simulink model "MissileMathSim"  (R2025a)
settings: Solver=ode4  StartTime=0.0  StopTime=inf  FixedStep=0.01  RelTol=1e-3
values from neighbouring files (symbols this model uses):
  phi00 = [0 0.5 1 1.5 2 2.5 3 3.5 4 4.5 5 5.5 ... (552 elements, 276x2)]    [pre-design_data.mat]
libraries: slpidlib x2, ASEToolBox x1, simulink x1
settings Model: Creator=admin  LastModifiedBy=zqhkd
settings DataIOCC: SaveFinalState=on  SaveOutput=off  InspectSignalLogs=on  SaveTime=off
settings OptimizationCC: DefaultParameterBehavior=Inlined  EnhancedBackFolding=on  PassReuseOutputArgsAs=Individual arguments  ZeroExternalMemoryAtStartup=off  ZeroInternalMemoryAtStartup=off  OptimizeBlockOrder=speed  DifferentSizesBufferReuse=on  OptimizationCustomize=off  EfficientTunableParamExpr=on
settings DebuggingCC: ParameterTunabilityLossMsg=error
settings HardwareCC: ProdBitPerLong=64.0  ProdHWDeviceType=Intel->x86-64 (Linux 64)
settings SFSimCC: MATLABDynamicMemAlloc=off
settings RTWCC: SystemTargetFile=ert.tlc  TemplateMakefile=ert_default_tmf  RetainRTWFile=on  Toolchain=Microsoft Visual C++ 2022 v17.0 | nmake (64-bit Windows)  GPUComputeCapability=3.5  Description=Embedded Coder
settings CodeAppCC: ForceParamTrailComments=on  IgnoreCustomStorageClasses=off  OperatorAnnotations=on  SimulinkDataObjDesc=on  SFDataObjDesc=on  InsertBlockDesc=on
settings ERTTargetCC: ExtModeTransport=0.0  ExtModeStaticAlloc=off  ExtModeMexFile=ext_comm  ExtModeIntrfLevel=Level1  ERTCustomFileTemplate=example_file_process.tlc  TargetLangStandard=C99 (ISO)  GenerateSampleERTMain=on

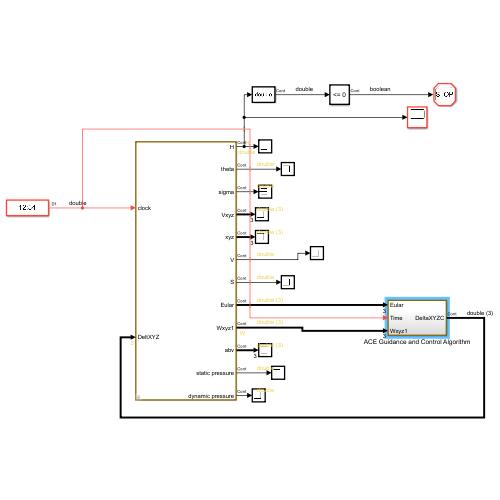
[thumbnail: Simulink's stored preview of the top-level diagram]
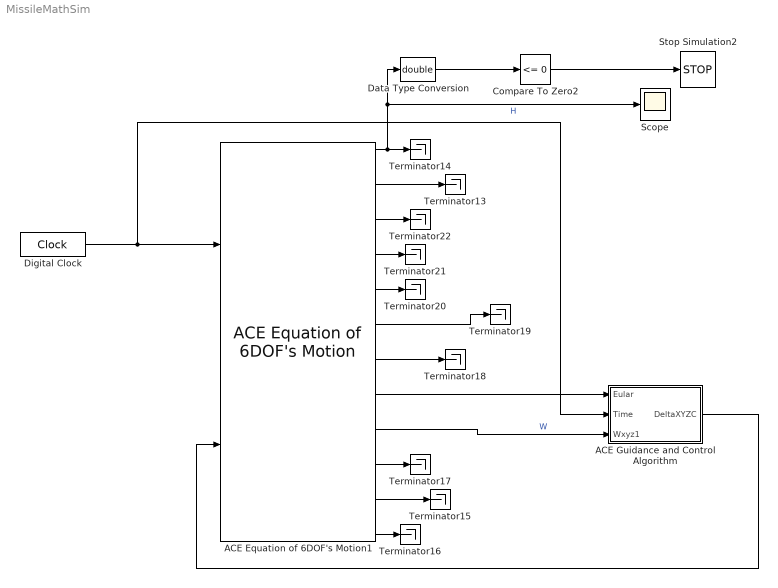
== system MissileMathSim ==
  ACE Equation of 6DOF's Motion1 : ASEToolBox/Aerocraft Model/ACE Equation of 6DOF's Motion
      settings: SourceProductName=ASEToolBox
  ACE Guidance and Control Algorithm : Subsystem
  Compare To Zero2 : simulink/Logic and Bit Operations/Compare To Zero  relop=<=  OutDataTypeStr=boolean
  Data Type Conversion : DataTypeConversion  OutDataTypeStr=double  SaturateOnIntegerOverflow=off  RndMeth=Floor
  Digital Clock : DigitalClock  SampleTime=0.01
  Scope : Scope
      settings: ActiveDisplayYMinimum=-113.65825705155464  ActiveDisplayYMaximum=1022.934313463992
  Stop Simulation2 : Stop
  Terminator{13..22} (10 alike) : Terminator
  wires:
  ACE Equation of 6DOF's Motion1/11 -> Terminator15/1
  ACE Equation of 6DOF's Motion1/3 -> Terminator22/1
  ACE Equation of 6DOF's Motion1/7 -> Terminator18/1
  ACE Equation of 6DOF's Motion1/8 -> ACE Guidance and Control Algorithm/1(Eular)
  ACE Equation of 6DOF's Motion1/2 -> Terminator13/1
  ACE Equation of 6DOF's Motion1/12 -> Terminator16/1
  ACE Equation of 6DOF's Motion1/1 -> Terminator14/1, Data Type Conversion/1, Scope/1  "H"
  ACE Equation of 6DOF's Motion1/4 -> Terminator21/1
  Compare To Zero2/1 -> Stop Simulation2/1
  ACE Equation of 6DOF's Motion1/6 -> Terminator19/1
  Digital Clock/1 -> ACE Guidance and Control Algorithm/2(Time), ACE Equation of 6DOF's Motion1/1
  ACE Equation of 6DOF's Motion1/5 -> Terminator20/1
  ACE Equation of 6DOF's Motion1/10 -> Terminator17/1
  ACE Guidance and Control Algorithm/1(DeltaXYZC) -> ACE Equation of 6DOF's Motion1/2
  Data Type Conversion/1 -> Compare To Zero2/1
  ACE Equation of 6DOF's Motion1/9 -> ACE Guidance and Control Algorithm/3(Wxyz1)  "W"

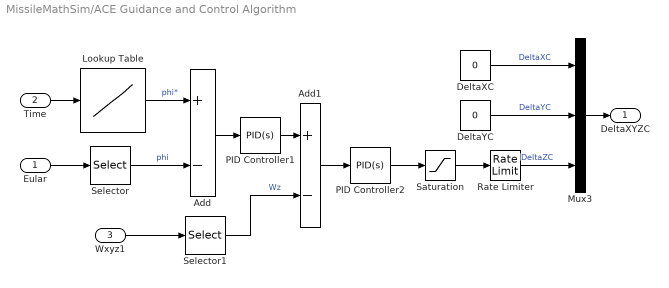
== system MissileMathSim/ACE Guidance and Control Algorithm ==
  Eular : Inport
  Time : Inport  Port=2
  Wxyz1 : Inport  Port=3
  Add : Sum  Inputs=+-
  Add1 : Sum  Inputs=+-
  DeltaXC : Constant  Value=0
  DeltaYC : Constant  Value=0
  Lookup Table : Lookup  InitFcn=|  InputValues=phi00(:,1)  Table=phi00(:,2)  SaturateOnIntegerOverflow=off
      | phi00=[0.0 	60
      | 0.5 	53.175
      | 1.0 	47.6
      | 1.5 	43.275
      | 2.0 	40.2
      | 2.5 	39.1055
      | 3.0 	38.012
      | 3.5 	36.9195
      | 4.0 	35.828
      | 4.5 	34.7375
      | 5.0 	33.648
      | 5.5 	32.5595
      | 6.0 	31.472
      | 6.5 	30.3855
      | 7.0 	29.3
      | 7.5 	28.2155
      | 8.0 	27.132
      | 8.5 	26.0495
      | 9.0 	24.968
      | 9.5 	23.8875
      | 10.0 	22.808
      | 10.5 	21.7295
      | 11.0 	20.652
      | 11.5 	19.5755
      | 12.0 	18.5
      | 12.5 	17.4255
      | 13.0 	16.352
      | 13.5 	15.2795
      | 14.0 	14.208
      | 14.5 	13.1375
      | 15.0 	12.068
      | 15.5 	10.9995
      | 16.0 	9.932
      | 16.5 	8.8655
      | 17.0 	7.8
      | 17.5 	6.7355
      | 18.0 	5.672
      | 18.5 	4.6095
      | 19.0 	3.548
      | 19.5 	2.4875
      | 20.0 	1.428
      | 20.5 	0.3695
      | 21.0 	-0.688
      | 21.5 	-1.7445
      | 22.0 	-2.8
      | 22.5 	-3.8545
      | 23.0 	-4.908
      | 23.5 	-5.9605
      | 24.0 	-7.012
      | 24.5 	-8.0625
      | 25.0 	-9.112
      | 25.5 	-10.1605
      | 26.0 	-11.208
      | 26.5 	-12.2545
      | 27.0 	-13.3
      | 27.5 	-14.3445
      | 28.0 	-15.388
      | 28.5 	-14.862975
      | 29.0 	-14.3379
      | 29.5 	-13.812775
      | 30.0 	-13.2876
      | 30.5 	-12.762375
      | 31.0 	-12.2371
      | 31.5 	-11.711775
      | 32.0 	-11.1864
      | 32.5 	-10.660975
      | 33.0 	-10.1355
      | 33.5 	-9.609975
      | 34.0 	-9.0844
      | 34.5 	-8.558775
      | 35.0 	-8.0331
      | 35.5 	-7.507375
      | 36.0 	-6.9816
      | 36.5 	-6.455775
      | 37.0 	-5.9299
      | 37.5 	-5.403975
      | 38.0 	-4.878
      | 38.5 	-4.351975
      | 39.0 	-3.8259
      | 39.5 	-3.299775
      | 40.0 	-2.7736
      | 40.5 	-2.247375
      | 41.0 	-1.7211
      | 41.5 	-1.194775
      | 42.0 	-0.6684
      | 42.5 	-0.141975
      | 43.0 	0.3845
      | 43.5 	0.911025
      | 44.0 	1.4376
      | 44.5 	1.964225
      | 45.0 	2.4909
      | 45.5 	3.0167
      | 46.0 	3.01485
      | 46.5 	3.0133
      | 47.0 	3.01205
      | 47.5 	3.0111
      | 48.0 	3.01045
      | 48.5 	3.0101
      | 49.0 	3.01005
      | 49.5 	3.0103
      | 50.0 	3.01085
      | 50.5 	3.0117
      | 51.0 	3.01285
      | 51.5 	3.0143
      | 52.0 	3.01605
      | 52.5 	3.0181
      | 53.0 	3.02045
      | 53.5 	3.0231
      | 54.0 	3.02605
      | 54.5 	3.0293
      | 55.0 	3.03285
      | 55.5 	3.0367
      | 56.0 	3.04085
      | 56.5 	3.0453
      | 57.0 	3.05005
      | 57.5 	3.0551
      | 58.0 	3.06045
      | 58.5 	3.0661
      | 59.0 	3.07205
      | 59.5 	3.0783
      | 60.0 	3.08485
      | 60.5 	3.0917
      | 61.0 	3.09885
      | 61.5 	3.1063
      | 62.0 	3.11405
      | 62.5 	3.1221
      | 63.0 	3.13045
      | 63.5 	3.1391
      | 64.0 	3.14805
      | 64.5 	3.1573
      | 65.0 	3.16685
      | 65.5 	3.1767
      | 66.0 	3.18685
      | 66.5 	3.1973
      | 67.0 	3.20805
      | 67.5 	3.2191
      | 68.0 	3.23045
      | 68.5 	3.2421
      | 69.0 	3.25405
      | 69.5 	3.2663
      | 70.0 	3.27885
      | 70.5 	3.2917
      | 71.0 	3.30485
      | 71.5 	3.3183
      | 72.0 	3.33205
      | 72.5 	3.3461
      | 73.0 	3.36045
      | 73.5 	3.3751
      | 74.0 	3.39005
      | 74.5 	3.4053
      | 75.0 	3.42085
      | 75.5 	3.4367
      | 76.0 	3.45285
      | 76.5 	3.4693
      | 77.0 	3.48605
      | 77.5 	3.5031
      | 78.0 	3.52045
      | 78.5 	3.5381
      | 79.0 	3.55605
      | 79.5 	3.5743
      | 80.0 	3.59285
      | 80.5 	3.6117
      | 81.0 	3.63085
      | 81.5 	3.6503
      | 82.0 	3.67005
      | 82.5 	3.6901
      | 83.0 	3.71045
      | 83.5 	3.7311
      | 84.0 	3.75205
      | 84.5 	3.7733
      | 85.0 	3.79485
      | 85.5 	3.8167
      | 86.0 	3.83885
      | 86.5 	3.8613
      | 87.0 	3.88405
      | 87.5 	3.9071
      | 88.0 	3.93045
      | 88.5 	3.9541
      | 89.0 	3.97805
      | 89.5 	4.0023
      | 90.0 	4.02685
      | 90.5 	4.0517
      | 91.0 	4.07685
      | 91.5 	4.1023
      | 92.0 	4.12805
      | 92.5 	4.1541
      | 93.0 	4.18045
      | 93.5 	4.2071
      | 94.0 	4.23405
      | 94.5 	4.2613
      | 95.0 	4.28885
      | 95.5 	4.3167
      | 96.0 	4.34485
      | 96.5 	4.3733
      | 97.0 	4.40205
      | 97.5 	4.4311
      | 98.0 	4.46045
      | 98.5 	4.4901
      | 99.0 	4.52005
      | 99.5 	4.5503
      | 100.0 	4.5808
      | 100.5 	5.4608
      | 101.0 	6.3008
      | 101.5 	7.1008
      | 102.0 	7.8608
      | 102.5 	8.5808
      | 103.0 	9.2608
      | 103.5 	9.9008
      | 104.0 	10.5008
      | 104.5 	11.0608
      | 105.0 	11.5808
      | 105.5 	12.0608
      | 106.0 	12.5008
      | 106.5 	12.9008
      | 107.0 	13.2608
      | 107.5 	13.5808
      | 108.0 	13.8608
      | 108.5 	14.1008
      | 109.0 	14.3008
      | 109.5 	14.4608
      | 110.0 	14.5808
      | 110.5 	14.6608
      | 111.0 	14.7008
      | 111.5 	14.7008
      | 112.0 	14.6608
      | 112.5 	14.5808
      | 113.0 	14.4608
      | 113.5 	14.3008
      | 114.0 	14.1008
      | 114.5 	13.8608
      | 115.0 	13.5808
      | 115.5 	13.2608
      | 116.0 	12.9008
      | 116.5 	12.5008
      | 117.0 	12.0608
      | 117.5 	11.5808
      | 118.0 	11.0608
      | 118.5 	10.5008
      | 119.0 	9.9008
      | 119.5 	9.2608
      | 120.0 	8.5808
      | 120.5 	7.8608
      | 121.0 	7.1008
      | 121.5 	6.3008
      | 122.0 	5.4608
      | 122.5 	4.5808
      | 123.0 	3.6608
      | 123.5 	2.7008
      | 124.0 	1.7008
      | 124.5 	0.6608
      | 125.0 	-0.4192
      | 125.5 	-1.5392
      | 126.0 	-2.6992
      | 126.5 	-3.8992
      | 127.0 	-5.1392
      | 127.5 	-6.4192
      | 128.0 	-7.7392
      | 128.5 	-9.0992
      | 129.0 	-10.4992
      | 129.5 	-11.9392
      | 130.0 	-13.4192
      | 130.5 	-14.9392
      | 131.0 	-16.4992
      | 131.5 	-18.0992
      | 132.0 	-19.7392
      | 132.5 	-21.4192
      | 133.0 	-23.1392
      | 133.5 	-24.8992
      | 134.0 	-26.6992
      | 134.5 	-28.5392
      | 135.0 	-30.4192
      | 135.5 	-32.3392
      | 136.0 	-34.2992
      | 136.5 	-36.2992
      | 137.0 	-38.3392
      | 137.5 	-40.4192];
  Mux3 : Mux  Inputs=3
  PID Controller1 : slpidlib/PID Controller  Controller=PID  Form=Parallel  TimeDomain=Continuous-time  UseExternalTs=off  SampleTime=-1  IntegratorMethod=Forward Euler  FilterMethod=Forward Euler  ControllerParametersSource=internal  P=3  I=0.0225  UseKiTs=off  D=0.0563  UseExternalDerivativeSource=off  N=100  UseFilter=on  TunerSelectOption=Transfer Function Based (PID Tuner App)  InitialConditionSource=internal  InitialConditionForIntegrator=0  InitialConditionForFilter=0  DifferentiatorICPrevScaledInput=0  ExternalReset=none  TrackingMode=off  Kt=1  LimitOutput=off  SatLimitsSource=internal  UpperSaturationLimit=inf  LowerSaturationLimit=-inf  LinearizeAsGain=off  AntiWindupMode=none  Kb=1  LimitIntegrator=off  UpperIntegratorSaturationLimit=inf  LowerIntegratorSaturationLimit=-inf  POutMin=[]  POutMax=[]  IOutMin=[]  IOutMax=[]  DOutMin=[]  DOutMax=[]  NOutMin=[]  NOutMax=[]  SumOutMin=[]  SumOutMax=[]  SaturationOutMin=[]  SaturationOutMax=[]  PParamMin=[]  PParamMax=[]  IParamMin=[]  IParamMax=[]  DParamMin=[]  DParamMax=[]  NParamMin=[]  NParamMax=[]  KbParamMin=[]  KbParamMax=[]  KtParamMin=[]  KtParamMax=[]  KbOutMin=[]  KbOutMax=[]  KtOutMin=[]  KtOutMax=[]  IntegratorOutMin=[]  IntegratorOutMax=[]  FilterOutMin=[]  FilterOutMax=[]  SumI1OutMin=[]  SumI1OutMax=[]  SumI2OutMin=[]  SumI2OutMax=[]  SumI3OutMin=[]  SumI3OutMax=[]  SumI4OutMin=[]  SumI4OutMax=[]  SumDOutMin=[]  SumDOutMax=[]  DifferentiatorOutMin=[]  DifferentiatorOutMax=[]  FilterDiffOutCoefMin=[]  FilterDiffOutCoefMax=[]  ReciprocalOutMin=[]  ReciprocalOutMax=[]  SumDenOutMin=[]  SumDenOutMax=[]  SumNumOutMin=[]  SumNumOutMax=[]  DivideOutMin=[]  DivideOutMax=[]  UdiffTsProdOutMin=[]  UdiffTsProdOutMax=[]  NTsProdOutMin=[]  NTsProdOutMax=[]  UintegralTsProdOutMin=[]  UintegralTsProdOutMax=[]  UngainTsProdOutMin=[]  UngainTsProdOutMax=[]  ClampingZeroOutDataTypeStr=Inherit: Inherit via back propagation  ClampingZeroOutMin=[]  ClampingZeroOutMax=[]  FilterDenConstantOutDataTypeStr=Inherit: Inherit via back propagation  FilterDenConstantOutMin=[]  FilterDenConstantOutMax=[]  PCopyOutDataTypeStr=Inherit: Inherit via back propagation  PCopyOutMin=[]  PCopyOutMax=[]  NCopyOutDataTypeStr=Inherit: Inherit via back propagation  NCopyOutMin=[]  NCopyOutMax=[]  IntegratorContinuousStateAttributes=''  IntegratorStateMustResolveToSignalObject=off  IntegratorRTWStateStorageClass=Auto  FilterContinuousStateAttributes=''  FilterStateMustResolveToSignalObject=off  FilterRTWStateStorageClass=Auto  ParallelPVariant=InternalParameters  IdealPVariant=Disabled  IVariant=InternalParameters  DVariant=InternalParameters  IntegratorVariant=Continuous  SatVariant=Disabled  AWVariant=Passthrough  PCopyVariant=Disabled  TRVariant=Disabled  FdbkBlocksVariant=Forward  IdealPFdbkVariant=Disabled  SatFdbkVariant=Disabled  DerivativeFilterVariant=ContFilter  NVariant=InternalParameters  NCopyVariant=Disabled  FilterICVariant=InternalICsFilter  IntegratorICVariant=InternalICs  ExternalResetVariant=Disabled  TRSumVariant=Passthrough  SumFdbkVariant=Disabled  SumVariant=Sum_PID  TsampFilterVariant=InternalTs  TsampNgainVariant=Passthrough  TsampIntegralVariant=Disabled_SignalSpec  ExternalSaturationOutDataTypeStr=Inherit: Same as second input  DerivativeSourceVariant=ErrorSignal  PreIntVariant=InternalPreInt
  PID Controller2 : slpidlib/PID Controller  Controller=PID  Form=Parallel  TimeDomain=Continuous-time  UseExternalTs=off  SampleTime=-1  IntegratorMethod=Forward Euler  FilterMethod=Forward Euler  ControllerParametersSource=internal  P=0.17  I=0.1  UseKiTs=off  D=0.01  UseExternalDerivativeSource=off  N=100  UseFilter=on  TunerSelectOption=Transfer Function Based (PID Tuner App)  InitialConditionSource=internal  InitialConditionForIntegrator=0  InitialConditionForFilter=0  DifferentiatorICPrevScaledInput=0  ExternalReset=none  TrackingMode=off  Kt=1  LimitOutput=off  SatLimitsSource=internal  UpperSaturationLimit=inf  LowerSaturationLimit=-inf  LinearizeAsGain=off  AntiWindupMode=none  Kb=1  LimitIntegrator=off  UpperIntegratorSaturationLimit=inf  LowerIntegratorSaturationLimit=-inf  POutMin=[]  POutMax=[]  IOutMin=[]  IOutMax=[]  DOutMin=[]  DOutMax=[]  NOutMin=[]  NOutMax=[]  SumOutMin=[]  SumOutMax=[]  SaturationOutMin=[]  SaturationOutMax=[]  PParamMin=[]  PParamMax=[]  IParamMin=[]  IParamMax=[]  DParamMin=[]  DParamMax=[]  NParamMin=[]  NParamMax=[]  KbParamMin=[]  KbParamMax=[]  KtParamMin=[]  KtParamMax=[]  KbOutMin=[]  KbOutMax=[]  KtOutMin=[]  KtOutMax=[]  IntegratorOutMin=[]  IntegratorOutMax=[]  FilterOutMin=[]  FilterOutMax=[]  SumI1OutMin=[]  SumI1OutMax=[]  SumI2OutMin=[]  SumI2OutMax=[]  SumI3OutMin=[]  SumI3OutMax=[]  SumI4OutMin=[]  SumI4OutMax=[]  SumDOutMin=[]  SumDOutMax=[]  DifferentiatorOutMin=[]  DifferentiatorOutMax=[]  FilterDiffOutCoefMin=[]  FilterDiffOutCoefMax=[]  ReciprocalOutMin=[]  ReciprocalOutMax=[]  SumDenOutMin=[]  SumDenOutMax=[]  SumNumOutMin=[]  SumNumOutMax=[]  DivideOutMin=[]  DivideOutMax=[]  UdiffTsProdOutMin=[]  UdiffTsProdOutMax=[]  NTsProdOutMin=[]  NTsProdOutMax=[]  UintegralTsProdOutMin=[]  UintegralTsProdOutMax=[]  UngainTsProdOutMin=[]  UngainTsProdOutMax=[]  ClampingZeroOutDataTypeStr=Inherit: Inherit via back propagation  ClampingZeroOutMin=[]  ClampingZeroOutMax=[]  FilterDenConstantOutDataTypeStr=Inherit: Inherit via back propagation  FilterDenConstantOutMin=[]  FilterDenConstantOutMax=[]  PCopyOutDataTypeStr=Inherit: Inherit via back propagation  PCopyOutMin=[]  PCopyOutMax=[]  NCopyOutDataTypeStr=Inherit: Inherit via back propagation  NCopyOutMin=[]  NCopyOutMax=[]  IntegratorContinuousStateAttributes=''  IntegratorStateMustResolveToSignalObject=off  IntegratorRTWStateStorageClass=Auto  FilterContinuousStateAttributes=''  FilterStateMustResolveToSignalObject=off  FilterRTWStateStorageClass=Auto  ParallelPVariant=InternalParameters  IdealPVariant=Disabled  IVariant=InternalParameters  DVariant=InternalParameters  IntegratorVariant=Continuous  SatVariant=Disabled  AWVariant=Passthrough  PCopyVariant=Disabled  TRVariant=Disabled  FdbkBlocksVariant=Forward  IdealPFdbkVariant=Disabled  SatFdbkVariant=Disabled  DerivativeFilterVariant=ContFilter  NVariant=InternalParameters  NCopyVariant=Disabled  FilterICVariant=InternalICsFilter  IntegratorICVariant=InternalICs  ExternalResetVariant=Disabled  TRSumVariant=Passthrough  SumFdbkVariant=Disabled  SumVariant=Sum_PID  TsampFilterVariant=InternalTs  TsampNgainVariant=Passthrough  TsampIntegralVariant=Disabled_SignalSpec  ExternalSaturationOutDataTypeStr=Inherit: Same as second input  DerivativeSourceVariant=ErrorSignal  PreIntVariant=InternalPreInt
  Rate Limiter : RateLimiter  RisingSlewLimit=100  FallingSlewLimit=-100  SampleTimeMode=inherited
  Saturation : Saturate  UpperLimit=15  LowerLimit=-15
  Selector : Selector  InputPortWidth=3  IndexOptions=Index vector (dialog)  Indices=1  OutputSizes=1
  Selector1 : Selector  InputPortWidth=3  IndexOptions=Index vector (dialog)  Indices=3  OutputSizes=1
  DeltaXYZC : Outport
  wires:
  Rate Limiter/1 -> Mux3/3  "DeltaZC"
  Saturation/1 -> Rate Limiter/1
  PID Controller2/1 -> Saturation/1
  Selector/1 -> Add/2  "phi"
  DeltaXC/1 -> Mux3/1  "DeltaXC"
  DeltaYC/1 -> Mux3/2  "DeltaYC"
  Eular/1 -> Selector/1
  Lookup Table/1 -> Add/1  "phi*"
  Time/1 -> Lookup Table/1
  Mux3/1 -> DeltaXYZC/1
  Wxyz1/1 -> Selector1/1
  Add/1 -> PID Controller1/1
  Add1/1 -> PID Controller2/1
  Selector1/1 -> Add1/2  "Wz"
  PID Controller1/1 -> Add1/1
